simulink library "lib_SecCtrl_MASmsg"  (R2026a)
settings: Solver=VariableStepAuto
undefined symbols (not defined in the file): buses_lf, DiscIntNeverNeededParam, entity, iPs_lf, iQs_lf, last_send, m, Ps_lf, Qs_lf, set_DG_up, set_extra_satur, set_sending_cost, v_buses_mod
libraries: simulink x400, sl_discontinuities x10, eeGeneralControl x5
(part 9 of 12)

== system lib_SecCtrl_MASmsg/MAS messages/ID1/Send to neighbor1/five ==
  Message : Inport
  Cast1 : EntityMulticast  InputPortMessageModes=m  MulticastTag=ID2
  Cast1all : EntityMulticast  InputPortMessageModes=m  MulticastTag=ID2
  Cast2 : EntityMulticast  InputPortMessageModes=m  MulticastTag=ID2
  Cast2all : EntityMulticast  InputPortMessageModes=m  MulticastTag=ID2
  Cast3 : EntityMulticast  InputPortMessageModes=m  MulticastTag=ID0
  Cast3all : EntityMulticast  InputPortMessageModes=m  MulticastTag=ID0
  Cast4 : EntityMulticast  InputPortMessageModes=m  MulticastTag=ID0
  Cast4all : EntityMulticast  InputPortMessageModes=m  MulticastTag=ID0
  Cast5 : EntityMulticast  InputPortMessageModes=m  MulticastTag=ID0
  Cast5all : EntityMulticast  InputPortMessageModes=m  MulticastTag=ID0
  Entity Output Switch : EntityOutputSwitch  InputPortMessageModes=m  OutputPortMessageModes=m,m,m,m,m,m  NumberOutputPorts=6  SwitchingCriterion=From attribute  SwitchAttributeName=Select  InitialPortSelection=3
      settings: OutputPortMap=o0,o1,o2,o3,o4,o5
  Entity Replicator1 : EntityReplicator  InputPortMessageModes=m  OutputPortMessageModes=m,m,m,m,m  NumberReplicas=4
      settings: OutputPortMap=o0,o1,o2,o3,o4
  Entity Server : EntityServer  InputPortMessageModes=m  OutputPortMessageModes=m  Capacity=1  ServiceTimeValue=0  EntryAction=entity.Select = select(entity.Dest);
  select : Subsystem  TreatAsAtomicUnit=on
  wires:
  Entity Server/1 -> Entity Output Switch/1
  Entity Output Switch/5 -> Cast5/1
  Entity Output Switch/1 -> Cast1/1
  Entity Replicator1/3 -> Cast3all/1
  Entity Replicator1/4 -> Cast4all/1
  Entity Output Switch/3 -> Cast3/1
  Entity Output Switch/2 -> Cast2/1
  Entity Replicator1/2 -> Cast2all/1
  Entity Replicator1/1 -> Cast1all/1
  Message/1 -> Entity Server/1  "Message"
  Entity Replicator1/5 -> Cast5all/1
  Entity Output Switch/6 -> Entity Replicator1/1
  Entity Output Switch/4 -> Cast4/1

== system lib_SecCtrl_MASmsg/MAS messages/ID1/Send to neighbor1/four ==
  Message : Inport
  Cast1 : EntityMulticast  InputPortMessageModes=m  MulticastTag=ID1
  Cast1all : EntityMulticast  InputPortMessageModes=m  MulticastTag=ID1
  Cast2 : EntityMulticast  InputPortMessageModes=m  MulticastTag=ID3
  Cast2all : EntityMulticast  InputPortMessageModes=m  MulticastTag=ID3
  Cast3 : EntityMulticast  InputPortMessageModes=m  MulticastTag=ID0
  Cast3all : EntityMulticast  InputPortMessageModes=m  MulticastTag=ID0
  Cast4 : EntityMulticast  InputPortMessageModes=m  MulticastTag=ID0
  Cast4all : EntityMulticast  InputPortMessageModes=m  MulticastTag=ID0
  Entity Output Switch : EntityOutputSwitch  InputPortMessageModes=m  OutputPortMessageModes=m,m,m,m,m  NumberOutputPorts=5  SwitchingCriterion=From attribute  SwitchAttributeName=Select  InitialPortSelection=3
      settings: OutputPortMap=o0,o1,o2,o3,o4
  Entity Replicator1 : EntityReplicator  InputPortMessageModes=m  OutputPortMessageModes=m,m,m,m  NumberReplicas=3
      settings: OutputPortMap=o0,o1,o2,o3
  Entity Server : EntityServer  InputPortMessageModes=m  OutputPortMessageModes=m  Capacity=1  ServiceTimeValue=0  EntryAction=entity.Select = select(entity.Dest);
  select : Subsystem  TreatAsAtomicUnit=on
  wires:
  Entity Server/1 -> Entity Output Switch/1
  Message/1 -> Entity Server/1  "Message"
  Entity Output Switch/4 -> Cast4/1
  Entity Output Switch/2 -> Cast2/1
  Entity Replicator1/2 -> Cast2all/1
  Entity Replicator1/1 -> Cast1all/1
  Entity Output Switch/1 -> Cast1/1
  Entity Output Switch/3 -> Cast3/1
  Entity Output Switch/5 -> Entity Replicator1/1
  Entity Replicator1/4 -> Cast4all/1
  Entity Replicator1/3 -> Cast3all/1

== system lib_SecCtrl_MASmsg/MAS messages/ID1/Send to neighbor1/one ==
  Message : Inport
  Cast : EntityMulticast  InputPortMessageModes=m  MulticastTag=ID2
  Castall : EntityMulticast  InputPortMessageModes=m  MulticastTag=ID2
  Entity Output Switch1 : EntityOutputSwitch  InputPortMessageModes=m  OutputPortMessageModes=m,m  SwitchingCriterion=From attribute  SwitchAttributeName=Select  InitialPortSelection=3
  Entity Server : EntityServer  InputPortMessageModes=m  OutputPortMessageModes=m  Capacity=1  ServiceTimeValue=0  EntryAction=entity.Select = select(entity.Dest);
  select : Subsystem  TreatAsAtomicUnit=on
  wires:
  Message/1 -> Entity Server/1  "Message"
  Entity Server/1 -> Entity Output Switch1/1
  Entity Output Switch1/1 -> Cast/1
  Entity Output Switch1/2 -> Castall/1

== system lib_SecCtrl_MASmsg/MAS messages/ID1/Send to neighbor1/three ==
  Message : Inport
  Cast1 : EntityMulticast  InputPortMessageModes=m  MulticastTag=ID0
  Cast1all : EntityMulticast  InputPortMessageModes=m  MulticastTag=ID0
  Cast2 : EntityMulticast  InputPortMessageModes=m  MulticastTag=ID0
  Cast2all : EntityMulticast  InputPortMessageModes=m  MulticastTag=ID0
  Cast3 : EntityMulticast  InputPortMessageModes=m  MulticastTag=ID0
  Cast3all : EntityMulticast  InputPortMessageModes=m  MulticastTag=ID0
  Entity Output Switch : EntityOutputSwitch  InputPortMessageModes=m  OutputPortMessageModes=m,m,m,m  NumberOutputPorts=4  SwitchingCriterion=From attribute  SwitchAttributeName=Select  InitialPortSelection=3
      settings: OutputPortMap=o0,o1,o2,o3
  Entity Replicator1 : EntityReplicator  InputPortMessageModes=m  OutputPortMessageModes=m,m,m  NumberReplicas=2
      settings: OutputPortMap=o0,o1,o2
  Entity Server : EntityServer  InputPortMessageModes=m  OutputPortMessageModes=m  Capacity=1  ServiceTimeValue=0  EntryAction=entity.Select = select(entity.Dest);
  select : Subsystem  TreatAsAtomicUnit=on
  wires:
  Entity Server/1 -> Entity Output Switch/1
  Message/1 -> Entity Server/1  "Message"
  Entity Output Switch/3 -> Cast3/1
  Entity Replicator1/3 -> Cast3all/1
  Entity Output Switch/1 -> Cast1/1
  Entity Replicator1/1 -> Cast1all/1
  Entity Replicator1/2 -> Cast2all/1
  Entity Output Switch/2 -> Cast2/1
  Entity Output Switch/4 -> Entity Replicator1/1

== system lib_SecCtrl_MASmsg/MAS messages/ID1/Send to neighbor1/two ==
  Message : Inport
  Cast1 : EntityMulticast  InputPortMessageModes=m  MulticastTag=ID5
  Cast1all : EntityMulticast  InputPortMessageModes=m  MulticastTag=ID5
  Cast2 : EntityMulticast  InputPortMessageModes=m  MulticastTag=ID2
  Cast2all : EntityMulticast  InputPortMessageModes=m  MulticastTag=ID2
  Entity Output Switch : EntityOutputSwitch  InputPortMessageModes=m  OutputPortMessageModes=m,m,m  NumberOutputPorts=3  SwitchingCriterion=From attribute  SwitchAttributeName=Select  InitialPortSelection=3
      settings: OutputPortMap=o0,o1,o2
  Entity Replicator1 : EntityReplicator  InputPortMessageModes=m  OutputPortMessageModes=m,m
  Entity Server : EntityServer  InputPortMessageModes=m  OutputPortMessageModes=m  Capacity=1  ServiceTimeValue=0  EntryAction=entity.Select = select(entity.Dest);
  select : Subsystem  TreatAsAtomicUnit=on
  wires:
  Entity Server/1 -> Entity Output Switch/1
  Entity Output Switch/2 -> Cast2/1
  Entity Output Switch/1 -> Cast1/1
  Message/1 -> Entity Server/1  "Message"
  Entity Replicator1/1 -> Cast1all/1
  Entity Replicator1/2 -> Cast2all/1
  Entity Output Switch/3 -> Entity Replicator1/1

== system lib_SecCtrl_MASmsg/MAS messages/ID1/Send to neighbor2/five ==
  Message : Inport
  Cast1 : EntityMulticast  InputPortMessageModes=m  MulticastTag=ID2
  Cast1all : EntityMulticast  InputPortMessageModes=m  MulticastTag=ID2
  Cast2 : EntityMulticast  InputPortMessageModes=m  MulticastTag=ID2
  Cast2all : EntityMulticast  InputPortMessageModes=m  MulticastTag=ID2
  Cast3 : EntityMulticast  InputPortMessageModes=m  MulticastTag=ID0
  Cast3all : EntityMulticast  InputPortMessageModes=m  MulticastTag=ID0
  Cast4 : EntityMulticast  InputPortMessageModes=m  MulticastTag=ID0
  Cast4all : EntityMulticast  InputPortMessageModes=m  MulticastTag=ID0
  Cast5 : EntityMulticast  InputPortMessageModes=m  MulticastTag=ID0
  Cast5all : EntityMulticast  InputPortMessageModes=m  MulticastTag=ID0
  Entity Output Switch : EntityOutputSwitch  InputPortMessageModes=m  OutputPortMessageModes=m,m,m,m,m,m  NumberOutputPorts=6  SwitchingCriterion=From attribute  SwitchAttributeName=Select  InitialPortSelection=3
      settings: OutputPortMap=o0,o1,o2,o3,o4,o5
  Entity Replicator1 : EntityReplicator  InputPortMessageModes=m  OutputPortMessageModes=m,m,m,m,m  NumberReplicas=4
      settings: OutputPortMap=o0,o1,o2,o3,o4
  Entity Server : EntityServer  InputPortMessageModes=m  OutputPortMessageModes=m  Capacity=1  ServiceTimeValue=0  EntryAction=entity.Select = select(entity.Dest);
  select : Subsystem  TreatAsAtomicUnit=on
  wires:
  Entity Output Switch/4 -> Cast4/1
  Entity Output Switch/6 -> Entity Replicator1/1
  Entity Replicator1/5 -> Cast5all/1
  Message/1 -> Entity Server/1  "Message"
  Entity Replicator1/1 -> Cast1all/1
  Entity Replicator1/2 -> Cast2all/1
  Entity Output Switch/2 -> Cast2/1
  Entity Output Switch/3 -> Cast3/1
  Entity Replicator1/4 -> Cast4all/1
  Entity Replicator1/3 -> Cast3all/1
  Entity Output Switch/1 -> Cast1/1
  Entity Output Switch/5 -> Cast5/1
  Entity Server/1 -> Entity Output Switch/1

== system lib_SecCtrl_MASmsg/MAS messages/ID1/Send to neighbor2/four ==
  Message : Inport
  Cast1 : EntityMulticast  InputPortMessageModes=m  MulticastTag=ID1
  Cast1all : EntityMulticast  InputPortMessageModes=m  MulticastTag=ID1
  Cast2 : EntityMulticast  InputPortMessageModes=m  MulticastTag=ID3
  Cast2all : EntityMulticast  InputPortMessageModes=m  MulticastTag=ID3
  Cast3 : EntityMulticast  InputPortMessageModes=m  MulticastTag=ID0
  Cast3all : EntityMulticast  InputPortMessageModes=m  MulticastTag=ID0
  Cast4 : EntityMulticast  InputPortMessageModes=m  MulticastTag=ID0
  Cast4all : EntityMulticast  InputPortMessageModes=m  MulticastTag=ID0
  Entity Output Switch : EntityOutputSwitch  InputPortMessageModes=m  OutputPortMessageModes=m,m,m,m,m  NumberOutputPorts=5  SwitchingCriterion=From attribute  SwitchAttributeName=Select  InitialPortSelection=3
      settings: OutputPortMap=o0,o1,o2,o3,o4
  Entity Replicator1 : EntityReplicator  InputPortMessageModes=m  OutputPortMessageModes=m,m,m,m  NumberReplicas=3
      settings: OutputPortMap=o0,o1,o2,o3
  Entity Server : EntityServer  InputPortMessageModes=m  OutputPortMessageModes=m  Capacity=1  ServiceTimeValue=0  EntryAction=entity.Select = select(entity.Dest);
  select : Subsystem  TreatAsAtomicUnit=on
  wires:
  Entity Replicator1/3 -> Cast3all/1
  Entity Replicator1/4 -> Cast4all/1
  Entity Output Switch/5 -> Entity Replicator1/1
  Entity Output Switch/3 -> Cast3/1
  Entity Output Switch/1 -> Cast1/1
  Entity Replicator1/1 -> Cast1all/1
  Entity Replicator1/2 -> Cast2all/1
  Entity Output Switch/2 -> Cast2/1
  Entity Output Switch/4 -> Cast4/1
  Message/1 -> Entity Server/1  "Message"
  Entity Server/1 -> Entity Output Switch/1

== system lib_SecCtrl_MASmsg/MAS messages/ID1/Send to neighbor2/one ==
  Message : Inport
  Cast : EntityMulticast  InputPortMessageModes=m  MulticastTag=ID2
  Castall : EntityMulticast  InputPortMessageModes=m  MulticastTag=ID2
  Entity Output Switch1 : EntityOutputSwitch  InputPortMessageModes=m  OutputPortMessageModes=m,m  SwitchingCriterion=From attribute  SwitchAttributeName=Select  InitialPortSelection=3
  Entity Server : EntityServer  InputPortMessageModes=m  OutputPortMessageModes=m  Capacity=1  ServiceTimeValue=0  EntryAction=entity.Select = select(entity.Dest);
  select : Subsystem  TreatAsAtomicUnit=on
  wires:
  Entity Output Switch1/2 -> Castall/1
  Entity Output Switch1/1 -> Cast/1
  Entity Server/1 -> Entity Output Switch1/1
  Message/1 -> Entity Server/1  "Message"

== system lib_SecCtrl_MASmsg/MAS messages/ID1/Send to neighbor2/three ==
  Message : Inport
  Cast1 : EntityMulticast  InputPortMessageModes=m  MulticastTag=ID0
  Cast1all : EntityMulticast  InputPortMessageModes=m  MulticastTag=ID0
  Cast2 : EntityMulticast  InputPortMessageModes=m  MulticastTag=ID0
  Cast2all : EntityMulticast  InputPortMessageModes=m  MulticastTag=ID0
  Cast3 : EntityMulticast  InputPortMessageModes=m  MulticastTag=ID0
  Cast3all : EntityMulticast  InputPortMessageModes=m  MulticastTag=ID0
  Entity Output Switch : EntityOutputSwitch  InputPortMessageModes=m  OutputPortMessageModes=m,m,m,m  NumberOutputPorts=4  SwitchingCriterion=From attribute  SwitchAttributeName=Select  InitialPortSelection=3
      settings: OutputPortMap=o0,o1,o2,o3
  Entity Replicator1 : EntityReplicator  InputPortMessageModes=m  OutputPortMessageModes=m,m,m  NumberReplicas=2
      settings: OutputPortMap=o0,o1,o2
  Entity Server : EntityServer  InputPortMessageModes=m  OutputPortMessageModes=m  Capacity=1  ServiceTimeValue=0  EntryAction=entity.Select = select(entity.Dest);
  select : Subsystem  TreatAsAtomicUnit=on
  wires:
  Entity Output Switch/4 -> Entity Replicator1/1
  Entity Output Switch/2 -> Cast2/1
  Entity Replicator1/2 -> Cast2all/1
  Entity Replicator1/1 -> Cast1all/1
  Entity Output Switch/1 -> Cast1/1
  Entity Replicator1/3 -> Cast3all/1
  Entity Output Switch/3 -> Cast3/1
  Message/1 -> Entity Server/1  "Message"
  Entity Server/1 -> Entity Output Switch/1

== system lib_SecCtrl_MASmsg/MAS messages/ID1/Send to neighbor2/two ==
  Message : Inport
  Cast1 : EntityMulticast  InputPortMessageModes=m  MulticastTag=ID5
  Cast1all : EntityMulticast  InputPortMessageModes=m  MulticastTag=ID5
  Cast2 : EntityMulticast  InputPortMessageModes=m  MulticastTag=ID2
  Cast2all : EntityMulticast  InputPortMessageModes=m  MulticastTag=ID2
  Entity Output Switch : EntityOutputSwitch  InputPortMessageModes=m  OutputPortMessageModes=m,m,m  NumberOutputPorts=3  SwitchingCriterion=From attribute  SwitchAttributeName=Select  InitialPortSelection=3
      settings: OutputPortMap=o0,o1,o2
  Entity Replicator1 : EntityReplicator  InputPortMessageModes=m  OutputPortMessageModes=m,m
  Entity Server : EntityServer  InputPortMessageModes=m  OutputPortMessageModes=m  Capacity=1  ServiceTimeValue=0  EntryAction=entity.Select = select(entity.Dest);
  select : Subsystem  TreatAsAtomicUnit=on
  wires:
  Entity Output Switch/3 -> Entity Replicator1/1
  Entity Replicator1/2 -> Cast2all/1
  Entity Replicator1/1 -> Cast1all/1
  Message/1 -> Entity Server/1  "Message"
  Entity Output Switch/1 -> Cast1/1
  Entity Output Switch/2 -> Cast2/1
  Entity Server/1 -> Entity Output Switch/1

== system lib_SecCtrl_MASmsg/MAS messages/ID2/Send to neighbor/five ==
  Message : Inport
  Cast1 : EntityMulticast  InputPortMessageModes=m  MulticastTag=ID2
  Cast1all : EntityMulticast  InputPortMessageModes=m  MulticastTag=ID2
  Cast2 : EntityMulticast  InputPortMessageModes=m  MulticastTag=ID2
  Cast2all : EntityMulticast  InputPortMessageModes=m  MulticastTag=ID2
  Cast3 : EntityMulticast  InputPortMessageModes=m  MulticastTag=ID0
  Cast3all : EntityMulticast  InputPortMessageModes=m  MulticastTag=ID0
  Cast4 : EntityMulticast  InputPortMessageModes=m  MulticastTag=ID0
  Cast4all : EntityMulticast  InputPortMessageModes=m  MulticastTag=ID0
  Cast5 : EntityMulticast  InputPortMessageModes=m  MulticastTag=ID0
  Cast5all : EntityMulticast  InputPortMessageModes=m  MulticastTag=ID0
  Entity Output Switch : EntityOutputSwitch  InputPortMessageModes=m  OutputPortMessageModes=m,m,m,m,m,m  NumberOutputPorts=6  SwitchingCriterion=From attribute  SwitchAttributeName=Select  InitialPortSelection=3
      settings: OutputPortMap=o0,o1,o2,o3,o4,o5
  Entity Replicator1 : EntityReplicator  InputPortMessageModes=m  OutputPortMessageModes=m,m,m,m,m  NumberReplicas=4
      settings: OutputPortMap=o0,o1,o2,o3,o4
  Entity Server : EntityServer  InputPortMessageModes=m  OutputPortMessageModes=m  Capacity=1  ServiceTimeValue=0  EntryAction=entity.Select = select(entity.Dest);
  select : Subsystem  TreatAsAtomicUnit=on
  wires:
  Entity Server/1 -> Entity Output Switch/1
  Entity Output Switch/5 -> Cast5/1
  Entity Output Switch/1 -> Cast1/1
  Entity Replicator1/3 -> Cast3all/1
  Entity Replicator1/4 -> Cast4all/1
  Entity Output Switch/3 -> Cast3/1
  Entity Output Switch/2 -> Cast2/1
  Entity Replicator1/2 -> Cast2all/1
  Entity Replicator1/1 -> Cast1all/1
  Message/1 -> Entity Server/1  "Message"
  Entity Replicator1/5 -> Cast5all/1
  Entity Output Switch/6 -> Entity Replicator1/1
  Entity Output Switch/4 -> Cast4/1

== system lib_SecCtrl_MASmsg/MAS messages/ID2/Send to neighbor/four ==
  Message : Inport
  Cast1 : EntityMulticast  InputPortMessageModes=m  MulticastTag=ID1
  Cast1all : EntityMulticast  InputPortMessageModes=m  MulticastTag=ID1
  Cast2 : EntityMulticast  InputPortMessageModes=m  MulticastTag=ID3
  Cast2all : EntityMulticast  InputPortMessageModes=m  MulticastTag=ID3
  Cast3 : EntityMulticast  InputPortMessageModes=m  MulticastTag=ID0
  Cast3all : EntityMulticast  InputPortMessageModes=m  MulticastTag=ID0
  Cast4 : EntityMulticast  InputPortMessageModes=m  MulticastTag=ID0
  Cast4all : EntityMulticast  InputPortMessageModes=m  MulticastTag=ID0
  Entity Output Switch : EntityOutputSwitch  InputPortMessageModes=m  OutputPortMessageModes=m,m,m,m,m  NumberOutputPorts=5  SwitchingCriterion=From attribute  SwitchAttributeName=Select  InitialPortSelection=3
      settings: OutputPortMap=o0,o1,o2,o3,o4
  Entity Replicator1 : EntityReplicator  InputPortMessageModes=m  OutputPortMessageModes=m,m,m,m  NumberReplicas=3
      settings: OutputPortMap=o0,o1,o2,o3
  Entity Server : EntityServer  InputPortMessageModes=m  OutputPortMessageModes=m  Capacity=1  ServiceTimeValue=0  EntryAction=entity.Select = select(entity.Dest);
  select : Subsystem  TreatAsAtomicUnit=on
  wires:
  Entity Server/1 -> Entity Output Switch/1
  Message/1 -> Entity Server/1  "Message"
  Entity Output Switch/4 -> Cast4/1
  Entity Output Switch/2 -> Cast2/1
  Entity Replicator1/2 -> Cast2all/1
  Entity Replicator1/1 -> Cast1all/1
  Entity Output Switch/1 -> Cast1/1
  Entity Output Switch/3 -> Cast3/1
  Entity Output Switch/5 -> Entity Replicator1/1
  Entity Replicator1/4 -> Cast4all/1
  Entity Replicator1/3 -> Cast3all/1

== system lib_SecCtrl_MASmsg/MAS messages/ID2/Send to neighbor/one ==
  Message : Inport
  Cast : EntityMulticast  InputPortMessageModes=m  MulticastTag=ID2
  Castall : EntityMulticast  InputPortMessageModes=m  MulticastTag=ID2
  Entity Output Switch1 : EntityOutputSwitch  InputPortMessageModes=m  OutputPortMessageModes=m,m  SwitchingCriterion=From attribute  SwitchAttributeName=Select  InitialPortSelection=3
  Entity Server : EntityServer  InputPortMessageModes=m  OutputPortMessageModes=m  Capacity=1  ServiceTimeValue=0  EntryAction=entity.Select = select(entity.Dest);
  select : Subsystem  TreatAsAtomicUnit=on
  wires:
  Message/1 -> Entity Server/1  "Message"
  Entity Server/1 -> Entity Output Switch1/1
  Entity Output Switch1/1 -> Cast/1
  Entity Output Switch1/2 -> Castall/1

== system lib_SecCtrl_MASmsg/MAS messages/ID2/Send to neighbor/three ==
  Message : Inport
  Cast1 : EntityMulticast  InputPortMessageModes=m  MulticastTag=ID0
  Cast1all : EntityMulticast  InputPortMessageModes=m  MulticastTag=ID0
  Cast2 : EntityMulticast  InputPortMessageModes=m  MulticastTag=ID0
  Cast2all : EntityMulticast  InputPortMessageModes=m  MulticastTag=ID0
  Cast3 : EntityMulticast  InputPortMessageModes=m  MulticastTag=ID0
  Cast3all : EntityMulticast  InputPortMessageModes=m  MulticastTag=ID0
  Entity Output Switch : EntityOutputSwitch  InputPortMessageModes=m  OutputPortMessageModes=m,m,m,m  NumberOutputPorts=4  SwitchingCriterion=From attribute  SwitchAttributeName=Select  InitialPortSelection=3
      settings: OutputPortMap=o0,o1,o2,o3
  Entity Replicator1 : EntityReplicator  InputPortMessageModes=m  OutputPortMessageModes=m,m,m  NumberReplicas=2
      settings: OutputPortMap=o0,o1,o2
  Entity Server : EntityServer  InputPortMessageModes=m  OutputPortMessageModes=m  Capacity=1  ServiceTimeValue=0  EntryAction=entity.Select = select(entity.Dest);
  select : Subsystem  TreatAsAtomicUnit=on
  wires:
  Entity Server/1 -> Entity Output Switch/1
  Message/1 -> Entity Server/1  "Message"
  Entity Output Switch/3 -> Cast3/1
  Entity Replicator1/3 -> Cast3all/1
  Entity Output Switch/1 -> Cast1/1
  Entity Replicator1/1 -> Cast1all/1
  Entity Replicator1/2 -> Cast2all/1
  Entity Output Switch/2 -> Cast2/1
  Entity Output Switch/4 -> Entity Replicator1/1

== system lib_SecCtrl_MASmsg/MAS messages/ID2/Send to neighbor/two ==
  Message : Inport
  Cast1 : EntityMulticast  InputPortMessageModes=m  MulticastTag=ID1
  Cast1all : EntityMulticast  InputPortMessageModes=m  MulticastTag=ID1
  Cast2 : EntityMulticast  InputPortMessageModes=m  MulticastTag=ID3
  Cast2all : EntityMulticast  InputPortMessageModes=m  MulticastTag=ID3
  Entity Output Switch : EntityOutputSwitch  InputPortMessageModes=m  OutputPortMessageModes=m,m,m  NumberOutputPorts=3  SwitchingCriterion=From attribute  SwitchAttributeName=Select  InitialPortSelection=3
      settings: OutputPortMap=o0,o1,o2
  Entity Replicator1 : EntityReplicator  InputPortMessageModes=m  OutputPortMessageModes=m,m
  Entity Server : EntityServer  InputPortMessageModes=m  OutputPortMessageModes=m  Capacity=1  ServiceTimeValue=0  EntryAction=entity.Select = select(entity.Dest);
  select : Subsystem  TreatAsAtomicUnit=on
  wires:
  Entity Server/1 -> Entity Output Switch/1
  Entity Output Switch/2 -> Cast2/1
  Entity Output Switch/1 -> Cast1/1
  Message/1 -> Entity Server/1  "Message"
  Entity Replicator1/1 -> Cast1all/1
  Entity Replicator1/2 -> Cast2all/1
  Entity Output Switch/3 -> Entity Replicator1/1

== system lib_SecCtrl_MASmsg/MAS messages/ID2/Send to neighbor1/five ==
  Message : Inport
  Cast1 : EntityMulticast  InputPortMessageModes=m  MulticastTag=ID2
  Cast1all : EntityMulticast  InputPortMessageModes=m  MulticastTag=ID2
  Cast2 : EntityMulticast  InputPortMessageModes=m  MulticastTag=ID2
  Cast2all : EntityMulticast  InputPortMessageModes=m  MulticastTag=ID2
  Cast3 : EntityMulticast  InputPortMessageModes=m  MulticastTag=ID0
  Cast3all : EntityMulticast  InputPortMessageModes=m  MulticastTag=ID0
  Cast4 : EntityMulticast  InputPortMessageModes=m  MulticastTag=ID0
  Cast4all : EntityMulticast  InputPortMessageModes=m  MulticastTag=ID0
  Cast5 : EntityMulticast  InputPortMessageModes=m  MulticastTag=ID0
  Cast5all : EntityMulticast  InputPortMessageModes=m  MulticastTag=ID0
  Entity Output Switch : EntityOutputSwitch  InputPortMessageModes=m  OutputPortMessageModes=m,m,m,m,m,m  NumberOutputPorts=6  SwitchingCriterion=From attribute  SwitchAttributeName=Select  InitialPortSelection=3
      settings: OutputPortMap=o0,o1,o2,o3,o4,o5
  Entity Replicator1 : EntityReplicator  InputPortMessageModes=m  OutputPortMessageModes=m,m,m,m,m  NumberReplicas=4
      settings: OutputPortMap=o0,o1,o2,o3,o4
  Entity Server : EntityServer  InputPortMessageModes=m  OutputPortMessageModes=m  Capacity=1  ServiceTimeValue=0  EntryAction=entity.Select = select(entity.Dest);
  select : Subsystem  TreatAsAtomicUnit=on
  wires:
  Entity Output Switch/4 -> Cast4/1
  Entity Output Switch/6 -> Entity Replicator1/1
  Entity Replicator1/5 -> Cast5all/1
  Message/1 -> Entity Server/1  "Message"
  Entity Replicator1/1 -> Cast1all/1
  Entity Replicator1/2 -> Cast2all/1
  Entity Output Switch/2 -> Cast2/1
  Entity Output Switch/3 -> Cast3/1
  Entity Replicator1/4 -> Cast4all/1
  Entity Replicator1/3 -> Cast3all/1
  Entity Output Switch/1 -> Cast1/1
  Entity Output Switch/5 -> Cast5/1
  Entity Server/1 -> Entity Output Switch/1

== system lib_SecCtrl_MASmsg/MAS messages/ID2/Send to neighbor1/four ==
  Message : Inport
  Cast1 : EntityMulticast  InputPortMessageModes=m  MulticastTag=ID1
  Cast1all : EntityMulticast  InputPortMessageModes=m  MulticastTag=ID1
  Cast2 : EntityMulticast  InputPortMessageModes=m  MulticastTag=ID3
  Cast2all : EntityMulticast  InputPortMessageModes=m  MulticastTag=ID3
  Cast3 : EntityMulticast  InputPortMessageModes=m  MulticastTag=ID0
  Cast3all : EntityMulticast  InputPortMessageModes=m  MulticastTag=ID0
  Cast4 : EntityMulticast  InputPortMessageModes=m  MulticastTag=ID0
  Cast4all : EntityMulticast  InputPortMessageModes=m  MulticastTag=ID0
  Entity Output Switch : EntityOutputSwitch  InputPortMessageModes=m  OutputPortMessageModes=m,m,m,m,m  NumberOutputPorts=5  SwitchingCriterion=From attribute  SwitchAttributeName=Select  InitialPortSelection=3
      settings: OutputPortMap=o0,o1,o2,o3,o4
  Entity Replicator1 : EntityReplicator  InputPortMessageModes=m  OutputPortMessageModes=m,m,m,m  NumberReplicas=3
      settings: OutputPortMap=o0,o1,o2,o3
  Entity Server : EntityServer  InputPortMessageModes=m  OutputPortMessageModes=m  Capacity=1  ServiceTimeValue=0  EntryAction=entity.Select = select(entity.Dest);
  select : Subsystem  TreatAsAtomicUnit=on
  wires:
  Entity Replicator1/3 -> Cast3all/1
  Entity Replicator1/4 -> Cast4all/1
  Entity Output Switch/5 -> Entity Replicator1/1
  Entity Output Switch/3 -> Cast3/1
  Entity Output Switch/1 -> Cast1/1
  Entity Replicator1/1 -> Cast1all/1
  Entity Replicator1/2 -> Cast2all/1
  Entity Output Switch/2 -> Cast2/1
  Entity Output Switch/4 -> Cast4/1
  Message/1 -> Entity Server/1  "Message"
  Entity Server/1 -> Entity Output Switch/1

== system lib_SecCtrl_MASmsg/MAS messages/ID2/Send to neighbor1/one ==
  Message : Inport
  Cast : EntityMulticast  InputPortMessageModes=m  MulticastTag=ID2
  Castall : EntityMulticast  InputPortMessageModes=m  MulticastTag=ID2
  Entity Output Switch1 : EntityOutputSwitch  InputPortMessageModes=m  OutputPortMessageModes=m,m  SwitchingCriterion=From attribute  SwitchAttributeName=Select  InitialPortSelection=3
  Entity Server : EntityServer  InputPortMessageModes=m  OutputPortMessageModes=m  Capacity=1  ServiceTimeValue=0  EntryAction=entity.Select = select(entity.Dest);
  select : Subsystem  TreatAsAtomicUnit=on
  wires:
  Entity Output Switch1/2 -> Castall/1
  Entity Output Switch1/1 -> Cast/1
  Entity Server/1 -> Entity Output Switch1/1
  Message/1 -> Entity Server/1  "Message"

== system lib_SecCtrl_MASmsg/MAS messages/ID2/Send to neighbor1/three ==
  Message : Inport
  Cast1 : EntityMulticast  InputPortMessageModes=m  MulticastTag=ID0
  Cast1all : EntityMulticast  InputPortMessageModes=m  MulticastTag=ID0
  Cast2 : EntityMulticast  InputPortMessageModes=m  MulticastTag=ID0
  Cast2all : EntityMulticast  InputPortMessageModes=m  MulticastTag=ID0
  Cast3 : EntityMulticast  InputPortMessageModes=m  MulticastTag=ID0
  Cast3all : EntityMulticast  InputPortMessageModes=m  MulticastTag=ID0
  Entity Output Switch : EntityOutputSwitch  InputPortMessageModes=m  OutputPortMessageModes=m,m,m,m  NumberOutputPorts=4  SwitchingCriterion=From attribute  SwitchAttributeName=Select  InitialPortSelection=3
      settings: OutputPortMap=o0,o1,o2,o3
  Entity Replicator1 : EntityReplicator  InputPortMessageModes=m  OutputPortMessageModes=m,m,m  NumberReplicas=2
      settings: OutputPortMap=o0,o1,o2
  Entity Server : EntityServer  InputPortMessageModes=m  OutputPortMessageModes=m  Capacity=1  ServiceTimeValue=0  EntryAction=entity.Select = select(entity.Dest);
  select : Subsystem  TreatAsAtomicUnit=on
  wires:
  Entity Output Switch/4 -> Entity Replicator1/1
  Entity Output Switch/2 -> Cast2/1
  Entity Replicator1/2 -> Cast2all/1
  Entity Replicator1/1 -> Cast1all/1
  Entity Output Switch/1 -> Cast1/1
  Entity Replicator1/3 -> Cast3all/1
  Entity Output Switch/3 -> Cast3/1
  Message/1 -> Entity Server/1  "Message"
  Entity Server/1 -> Entity Output Switch/1

== system lib_SecCtrl_MASmsg/MAS messages/ID2/Send to neighbor1/two ==
  Message : Inport
  Cast1 : EntityMulticast  InputPortMessageModes=m  MulticastTag=ID1
  Cast1all : EntityMulticast  InputPortMessageModes=m  MulticastTag=ID1
  Cast2 : EntityMulticast  InputPortMessageModes=m  MulticastTag=ID3
  Cast2all : EntityMulticast  InputPortMessageModes=m  MulticastTag=ID3
  Entity Output Switch : EntityOutputSwitch  InputPortMessageModes=m  OutputPortMessageModes=m,m,m  NumberOutputPorts=3  SwitchingCriterion=From attribute  SwitchAttributeName=Select  InitialPortSelection=3
      settings: OutputPortMap=o0,o1,o2
  Entity Replicator1 : EntityReplicator  InputPortMessageModes=m  OutputPortMessageModes=m,m
  Entity Server : EntityServer  InputPortMessageModes=m  OutputPortMessageModes=m  Capacity=1  ServiceTimeValue=0  EntryAction=entity.Select = select(entity.Dest);
  select : Subsystem  TreatAsAtomicUnit=on
  wires:
  Entity Output Switch/3 -> Entity Replicator1/1
  Entity Replicator1/2 -> Cast2all/1
  Entity Replicator1/1 -> Cast1all/1
  Message/1 -> Entity Server/1  "Message"
  Entity Output Switch/1 -> Cast1/1
  Entity Output Switch/2 -> Cast2/1
  Entity Server/1 -> Entity Output Switch/1

== system lib_SecCtrl_MASmsg/MAS messages/ID2/Send to neighbor2/five ==
  Message : Inport
  Cast1 : EntityMulticast  InputPortMessageModes=m  MulticastTag=ID2
  Cast1all : EntityMulticast  InputPortMessageModes=m  MulticastTag=ID2
  Cast2 : EntityMulticast  InputPortMessageModes=m  MulticastTag=ID2
  Cast2all : EntityMulticast  InputPortMessageModes=m  MulticastTag=ID2
  Cast3 : EntityMulticast  InputPortMessageModes=m  MulticastTag=ID0
  Cast3all : EntityMulticast  InputPortMessageModes=m  MulticastTag=ID0
  Cast4 : EntityMulticast  InputPortMessageModes=m  MulticastTag=ID0
  Cast4all : EntityMulticast  InputPortMessageModes=m  MulticastTag=ID0
  Cast5 : EntityMulticast  InputPortMessageModes=m  MulticastTag=ID0
  Cast5all : EntityMulticast  InputPortMessageModes=m  MulticastTag=ID0
  Entity Output Switch : EntityOutputSwitch  InputPortMessageModes=m  OutputPortMessageModes=m,m,m,m,m,m  NumberOutputPorts=6  SwitchingCriterion=From attribute  SwitchAttributeName=Select  InitialPortSelection=3
      settings: OutputPortMap=o0,o1,o2,o3,o4,o5
  Entity Replicator1 : EntityReplicator  InputPortMessageModes=m  OutputPortMessageModes=m,m,m,m,m  NumberReplicas=4
      settings: OutputPortMap=o0,o1,o2,o3,o4
  Entity Server : EntityServer  InputPortMessageModes=m  OutputPortMessageModes=m  Capacity=1  ServiceTimeValue=0  EntryAction=entity.Select = select(entity.Dest);
  select : Subsystem  TreatAsAtomicUnit=on
  wires:
  Entity Server/1 -> Entity Output Switch/1
  Entity Output Switch/5 -> Cast5/1
  Entity Output Switch/1 -> Cast1/1
  Entity Replicator1/3 -> Cast3all/1
  Entity Replicator1/4 -> Cast4all/1
  Entity Output Switch/3 -> Cast3/1
  Entity Output Switch/2 -> Cast2/1
  Entity Replicator1/2 -> Cast2all/1
  Entity Replicator1/1 -> Cast1all/1
  Message/1 -> Entity Server/1  "Message"
  Entity Replicator1/5 -> Cast5all/1
  Entity Output Switch/6 -> Entity Replicator1/1
  Entity Output Switch/4 -> Cast4/1

== system lib_SecCtrl_MASmsg/MAS messages/ID2/Send to neighbor2/four ==
  Message : Inport
  Cast1 : EntityMulticast  InputPortMessageModes=m  MulticastTag=ID1
  Cast1all : EntityMulticast  InputPortMessageModes=m  MulticastTag=ID1
  Cast2 : EntityMulticast  InputPortMessageModes=m  MulticastTag=ID3
  Cast2all : EntityMulticast  InputPortMessageModes=m  MulticastTag=ID3
  Cast3 : EntityMulticast  InputPortMessageModes=m  MulticastTag=ID0
  Cast3all : EntityMulticast  InputPortMessageModes=m  MulticastTag=ID0
  Cast4 : EntityMulticast  InputPortMessageModes=m  MulticastTag=ID0
  Cast4all : EntityMulticast  InputPortMessageModes=m  MulticastTag=ID0
  Entity Output Switch : EntityOutputSwitch  InputPortMessageModes=m  OutputPortMessageModes=m,m,m,m,m  NumberOutputPorts=5  SwitchingCriterion=From attribute  SwitchAttributeName=Select  InitialPortSelection=3
      settings: OutputPortMap=o0,o1,o2,o3,o4
  Entity Replicator1 : EntityReplicator  InputPortMessageModes=m  OutputPortMessageModes=m,m,m,m  NumberReplicas=3
      settings: OutputPortMap=o0,o1,o2,o3
  Entity Server : EntityServer  InputPortMessageModes=m  OutputPortMessageModes=m  Capacity=1  ServiceTimeValue=0  EntryAction=entity.Select = select(entity.Dest);
  select : Subsystem  TreatAsAtomicUnit=on
  wires:
  Entity Server/1 -> Entity Output Switch/1
  Message/1 -> Entity Server/1  "Message"
  Entity Output Switch/4 -> Cast4/1
  Entity Output Switch/2 -> Cast2/1
  Entity Replicator1/2 -> Cast2all/1
  Entity Replicator1/1 -> Cast1all/1
  Entity Output Switch/1 -> Cast1/1
  Entity Output Switch/3 -> Cast3/1
  Entity Output Switch/5 -> Entity Replicator1/1
  Entity Replicator1/4 -> Cast4all/1
  Entity Replicator1/3 -> Cast3all/1

== system lib_SecCtrl_MASmsg/MAS messages/ID2/Send to neighbor2/one ==
  Message : Inport
  Cast : EntityMulticast  InputPortMessageModes=m  MulticastTag=ID2
  Castall : EntityMulticast  InputPortMessageModes=m  MulticastTag=ID2
  Entity Output Switch1 : EntityOutputSwitch  InputPortMessageModes=m  OutputPortMessageModes=m,m  SwitchingCriterion=From attribute  SwitchAttributeName=Select  InitialPortSelection=3
  Entity Server : EntityServer  InputPortMessageModes=m  OutputPortMessageModes=m  Capacity=1  ServiceTimeValue=0  EntryAction=entity.Select = select(entity.Dest);
  select : Subsystem  TreatAsAtomicUnit=on
  wires:
  Message/1 -> Entity Server/1  "Message"
  Entity Server/1 -> Entity Output Switch1/1
  Entity Output Switch1/1 -> Cast/1
  Entity Output Switch1/2 -> Castall/1

== system lib_SecCtrl_MASmsg/MAS messages/ID2/Send to neighbor2/three ==
  Message : Inport
  Cast1 : EntityMulticast  InputPortMessageModes=m  MulticastTag=ID0
  Cast1all : EntityMulticast  InputPortMessageModes=m  MulticastTag=ID0
  Cast2 : EntityMulticast  InputPortMessageModes=m  MulticastTag=ID0
  Cast2all : EntityMulticast  InputPortMessageModes=m  MulticastTag=ID0
  Cast3 : EntityMulticast  InputPortMessageModes=m  MulticastTag=ID0
  Cast3all : EntityMulticast  InputPortMessageModes=m  MulticastTag=ID0
  Entity Output Switch : EntityOutputSwitch  InputPortMessageModes=m  OutputPortMessageModes=m,m,m,m  NumberOutputPorts=4  SwitchingCriterion=From attribute  SwitchAttributeName=Select  InitialPortSelection=3
      settings: OutputPortMap=o0,o1,o2,o3
  Entity Replicator1 : EntityReplicator  InputPortMessageModes=m  OutputPortMessageModes=m,m,m  NumberReplicas=2
      settings: OutputPortMap=o0,o1,o2
  Entity Server : EntityServer  InputPortMessageModes=m  OutputPortMessageModes=m  Capacity=1  ServiceTimeValue=0  EntryAction=entity.Select = select(entity.Dest);
  select : Subsystem  TreatAsAtomicUnit=on
  wires:
  Entity Server/1 -> Entity Output Switch/1
  Message/1 -> Entity Server/1  "Message"
  Entity Output Switch/3 -> Cast3/1
  Entity Replicator1/3 -> Cast3all/1
  Entity Output Switch/1 -> Cast1/1
  Entity Replicator1/1 -> Cast1all/1
  Entity Replicator1/2 -> Cast2all/1
  Entity Output Switch/2 -> Cast2/1
  Entity Output Switch/4 -> Entity Replicator1/1

== system lib_SecCtrl_MASmsg/MAS messages/ID2/Send to neighbor2/two ==
  Message : Inport
  Cast1 : EntityMulticast  InputPortMessageModes=m  MulticastTag=ID1
  Cast1all : EntityMulticast  InputPortMessageModes=m  MulticastTag=ID1
  Cast2 : EntityMulticast  InputPortMessageModes=m  MulticastTag=ID3
  Cast2all : EntityMulticast  InputPortMessageModes=m  MulticastTag=ID3
  Entity Output Switch : EntityOutputSwitch  InputPortMessageModes=m  OutputPortMessageModes=m,m,m  NumberOutputPorts=3  SwitchingCriterion=From attribute  SwitchAttributeName=Select  InitialPortSelection=3
      settings: OutputPortMap=o0,o1,o2
  Entity Replicator1 : EntityReplicator  InputPortMessageModes=m  OutputPortMessageModes=m,m
  Entity Server : EntityServer  InputPortMessageModes=m  OutputPortMessageModes=m  Capacity=1  ServiceTimeValue=0  EntryAction=entity.Select = select(entity.Dest);
  select : Subsystem  TreatAsAtomicUnit=on
  wires:
  Entity Server/1 -> Entity Output Switch/1
  Entity Output Switch/2 -> Cast2/1
  Entity Output Switch/1 -> Cast1/1
  Message/1 -> Entity Server/1  "Message"
  Entity Replicator1/1 -> Cast1all/1
  Entity Replicator1/2 -> Cast2all/1
  Entity Output Switch/3 -> Entity Replicator1/1

== system lib_SecCtrl_MASmsg/MAS messages/ID3/Send to neighbor/five ==
  Message : Inport
  Cast1 : EntityMulticast  InputPortMessageModes=m  MulticastTag=ID2
  Cast1all : EntityMulticast  InputPortMessageModes=m  MulticastTag=ID2
  Cast2 : EntityMulticast  InputPortMessageModes=m  MulticastTag=ID2
  Cast2all : EntityMulticast  InputPortMessageModes=m  MulticastTag=ID2
  Cast3 : EntityMulticast  InputPortMessageModes=m  MulticastTag=ID0
  Cast3all : EntityMulticast  InputPortMessageModes=m  MulticastTag=ID0
  Cast4 : EntityMulticast  InputPortMessageModes=m  MulticastTag=ID0
  Cast4all : EntityMulticast  InputPortMessageModes=m  MulticastTag=ID0
  Cast5 : EntityMulticast  InputPortMessageModes=m  MulticastTag=ID0
  Cast5all : EntityMulticast  InputPortMessageModes=m  MulticastTag=ID0
  Entity Output Switch : EntityOutputSwitch  InputPortMessageModes=m  OutputPortMessageModes=m,m,m,m,m,m  NumberOutputPorts=6  SwitchingCriterion=From attribute  SwitchAttributeName=Select  InitialPortSelection=3
      settings: OutputPortMap=o0,o1,o2,o3,o4,o5
  Entity Replicator1 : EntityReplicator  InputPortMessageModes=m  OutputPortMessageModes=m,m,m,m,m  NumberReplicas=4
      settings: OutputPortMap=o0,o1,o2,o3,o4
  Entity Server : EntityServer  InputPortMessageModes=m  OutputPortMessageModes=m  Capacity=1  ServiceTimeValue=0  EntryAction=entity.Select = select(entity.Dest);
  select : Subsystem  TreatAsAtomicUnit=on
  wires:
  Entity Server/1 -> Entity Output Switch/1
  Entity Output Switch/5 -> Cast5/1
  Entity Output Switch/1 -> Cast1/1
  Entity Replicator1/3 -> Cast3all/1
  Entity Replicator1/4 -> Cast4all/1
  Entity Output Switch/3 -> Cast3/1
  Entity Output Switch/2 -> Cast2/1
  Entity Replicator1/2 -> Cast2all/1
  Entity Replicator1/1 -> Cast1all/1
  Message/1 -> Entity Server/1  "Message"
  Entity Replicator1/5 -> Cast5all/1
  Entity Output Switch/6 -> Entity Replicator1/1
  Entity Output Switch/4 -> Cast4/1

== system lib_SecCtrl_MASmsg/MAS messages/ID3/Send to neighbor/four ==
  Message : Inport
  Cast1 : EntityMulticast  InputPortMessageModes=m  MulticastTag=ID1
  Cast1all : EntityMulticast  InputPortMessageModes=m  MulticastTag=ID1
  Cast2 : EntityMulticast  InputPortMessageModes=m  MulticastTag=ID3
  Cast2all : EntityMulticast  InputPortMessageModes=m  MulticastTag=ID3
  Cast3 : EntityMulticast  InputPortMessageModes=m  MulticastTag=ID0
  Cast3all : EntityMulticast  InputPortMessageModes=m  MulticastTag=ID0
  Cast4 : EntityMulticast  InputPortMessageModes=m  MulticastTag=ID0
  Cast4all : EntityMulticast  InputPortMessageModes=m  MulticastTag=ID0
  Entity Output Switch : EntityOutputSwitch  InputPortMessageModes=m  OutputPortMessageModes=m,m,m,m,m  NumberOutputPorts=5  SwitchingCriterion=From attribute  SwitchAttributeName=Select  InitialPortSelection=3
      settings: OutputPortMap=o0,o1,o2,o3,o4
  Entity Replicator1 : EntityReplicator  InputPortMessageModes=m  OutputPortMessageModes=m,m,m,m  NumberReplicas=3
      settings: OutputPortMap=o0,o1,o2,o3
  Entity Server : EntityServer  InputPortMessageModes=m  OutputPortMessageModes=m  Capacity=1  ServiceTimeValue=0  EntryAction=entity.Select = select(entity.Dest);
  select : Subsystem  TreatAsAtomicUnit=on
  wires:
  Entity Server/1 -> Entity Output Switch/1
  Message/1 -> Entity Server/1  "Message"
  Entity Output Switch/4 -> Cast4/1
  Entity Output Switch/2 -> Cast2/1
  Entity Replicator1/2 -> Cast2all/1
  Entity Replicator1/1 -> Cast1all/1
  Entity Output Switch/1 -> Cast1/1
  Entity Output Switch/3 -> Cast3/1
  Entity Output Switch/5 -> Entity Replicator1/1
  Entity Replicator1/4 -> Cast4all/1
  Entity Replicator1/3 -> Cast3all/1

== system lib_SecCtrl_MASmsg/MAS messages/ID3/Send to neighbor/one ==
  Message : Inport
  Cast : EntityMulticast  InputPortMessageModes=m  MulticastTag=ID2
  Castall : EntityMulticast  InputPortMessageModes=m  MulticastTag=ID2
  Entity Output Switch1 : EntityOutputSwitch  InputPortMessageModes=m  OutputPortMessageModes=m,m  SwitchingCriterion=From attribute  SwitchAttributeName=Select  InitialPortSelection=3
  Entity Server : EntityServer  InputPortMessageModes=m  OutputPortMessageModes=m  Capacity=1  ServiceTimeValue=0  EntryAction=entity.Select = select(entity.Dest);
  select : Subsystem  TreatAsAtomicUnit=on
  wires:
  Message/1 -> Entity Server/1  "Message"
  Entity Server/1 -> Entity Output Switch1/1
  Entity Output Switch1/1 -> Cast/1
  Entity Output Switch1/2 -> Castall/1

== system lib_SecCtrl_MASmsg/MAS messages/ID3/Send to neighbor/three ==
  Message : Inport
  Cast1 : EntityMulticast  InputPortMessageModes=m  MulticastTag=ID0
  Cast1all : EntityMulticast  InputPortMessageModes=m  MulticastTag=ID0
  Cast2 : EntityMulticast  InputPortMessageModes=m  MulticastTag=ID0
  Cast2all : EntityMulticast  InputPortMessageModes=m  MulticastTag=ID0
  Cast3 : EntityMulticast  InputPortMessageModes=m  MulticastTag=ID0
  Cast3all : EntityMulticast  InputPortMessageModes=m  MulticastTag=ID0
  Entity Output Switch : EntityOutputSwitch  InputPortMessageModes=m  OutputPortMessageModes=m,m,m,m  NumberOutputPorts=4  SwitchingCriterion=From attribute  SwitchAttributeName=Select  InitialPortSelection=3
      settings: OutputPortMap=o0,o1,o2,o3
  Entity Replicator1 : EntityReplicator  InputPortMessageModes=m  OutputPortMessageModes=m,m,m  NumberReplicas=2
      settings: OutputPortMap=o0,o1,o2
  Entity Server : EntityServer  InputPortMessageModes=m  OutputPortMessageModes=m  Capacity=1  ServiceTimeValue=0  EntryAction=entity.Select = select(entity.Dest);
  select : Subsystem  TreatAsAtomicUnit=on
  wires:
  Entity Server/1 -> Entity Output Switch/1
  Message/1 -> Entity Server/1  "Message"
  Entity Output Switch/3 -> Cast3/1
  Entity Replicator1/3 -> Cast3all/1
  Entity Output Switch/1 -> Cast1/1
  Entity Replicator1/1 -> Cast1all/1
  Entity Replicator1/2 -> Cast2all/1
  Entity Output Switch/2 -> Cast2/1
  Entity Output Switch/4 -> Entity Replicator1/1

== system lib_SecCtrl_MASmsg/MAS messages/ID3/Send to neighbor/two ==
  Message : Inport
  Cast1 : EntityMulticast  InputPortMessageModes=m  MulticastTag=ID2
  Cast1all : EntityMulticast  InputPortMessageModes=m  MulticastTag=ID2
  Cast2 : EntityMulticast  InputPortMessageModes=m  MulticastTag=ID4
  Cast2all : EntityMulticast  InputPortMessageModes=m  MulticastTag=ID4
  Entity Output Switch : EntityOutputSwitch  InputPortMessageModes=m  OutputPortMessageModes=m,m,m  NumberOutputPorts=3  SwitchingCriterion=From attribute  SwitchAttributeName=Select  InitialPortSelection=3
      settings: OutputPortMap=o0,o1,o2
  Entity Replicator1 : EntityReplicator  InputPortMessageModes=m  OutputPortMessageModes=m,m
  Entity Server : EntityServer  InputPortMessageModes=m  OutputPortMessageModes=m  Capacity=1  ServiceTimeValue=0  EntryAction=entity.Select = select(entity.Dest);
  select : Subsystem  TreatAsAtomicUnit=on
  wires:
  Entity Server/1 -> Entity Output Switch/1
  Entity Output Switch/2 -> Cast2/1
  Entity Output Switch/1 -> Cast1/1
  Message/1 -> Entity Server/1  "Message"
  Entity Replicator1/1 -> Cast1all/1
  Entity Replicator1/2 -> Cast2all/1
  Entity Output Switch/3 -> Entity Replicator1/1

== system lib_SecCtrl_MASmsg/MAS messages/ID3/Send to neighbor1/five ==
  Message : Inport
  Cast1 : EntityMulticast  InputPortMessageModes=m  MulticastTag=ID2
  Cast1all : EntityMulticast  InputPortMessageModes=m  MulticastTag=ID2
  Cast2 : EntityMulticast  InputPortMessageModes=m  MulticastTag=ID2
  Cast2all : EntityMulticast  InputPortMessageModes=m  MulticastTag=ID2
  Cast3 : EntityMulticast  InputPortMessageModes=m  MulticastTag=ID0
  Cast3all : EntityMulticast  InputPortMessageModes=m  MulticastTag=ID0
  Cast4 : EntityMulticast  InputPortMessageModes=m  MulticastTag=ID0
  Cast4all : EntityMulticast  InputPortMessageModes=m  MulticastTag=ID0
  Cast5 : EntityMulticast  InputPortMessageModes=m  MulticastTag=ID0
  Cast5all : EntityMulticast  InputPortMessageModes=m  MulticastTag=ID0
  Entity Output Switch : EntityOutputSwitch  InputPortMessageModes=m  OutputPortMessageModes=m,m,m,m,m,m  NumberOutputPorts=6  SwitchingCriterion=From attribute  SwitchAttributeName=Select  InitialPortSelection=3
      settings: OutputPortMap=o0,o1,o2,o3,o4,o5
  Entity Replicator1 : EntityReplicator  InputPortMessageModes=m  OutputPortMessageModes=m,m,m,m,m  NumberReplicas=4
      settings: OutputPortMap=o0,o1,o2,o3,o4
  Entity Server : EntityServer  InputPortMessageModes=m  OutputPortMessageModes=m  Capacity=1  ServiceTimeValue=0  EntryAction=entity.Select = select(entity.Dest);
  select : Subsystem  TreatAsAtomicUnit=on
  wires:
  Entity Output Switch/4 -> Cast4/1
  Entity Output Switch/6 -> Entity Replicator1/1
  Entity Replicator1/5 -> Cast5all/1
  Message/1 -> Entity Server/1  "Message"
  Entity Replicator1/1 -> Cast1all/1
  Entity Replicator1/2 -> Cast2all/1
  Entity Output Switch/2 -> Cast2/1
  Entity Output Switch/3 -> Cast3/1
  Entity Replicator1/4 -> Cast4all/1
  Entity Replicator1/3 -> Cast3all/1
  Entity Output Switch/1 -> Cast1/1
  Entity Output Switch/5 -> Cast5/1
  Entity Server/1 -> Entity Output Switch/1

== system lib_SecCtrl_MASmsg/MAS messages/ID3/Send to neighbor1/four ==
  Message : Inport
  Cast1 : EntityMulticast  InputPortMessageModes=m  MulticastTag=ID1
  Cast1all : EntityMulticast  InputPortMessageModes=m  MulticastTag=ID1
  Cast2 : EntityMulticast  InputPortMessageModes=m  MulticastTag=ID3
  Cast2all : EntityMulticast  InputPortMessageModes=m  MulticastTag=ID3
  Cast3 : EntityMulticast  InputPortMessageModes=m  MulticastTag=ID0
  Cast3all : EntityMulticast  InputPortMessageModes=m  MulticastTag=ID0
  Cast4 : EntityMulticast  InputPortMessageModes=m  MulticastTag=ID0
  Cast4all : EntityMulticast  InputPortMessageModes=m  MulticastTag=ID0
  Entity Output Switch : EntityOutputSwitch  InputPortMessageModes=m  OutputPortMessageModes=m,m,m,m,m  NumberOutputPorts=5  SwitchingCriterion=From attribute  SwitchAttributeName=Select  InitialPortSelection=3
      settings: OutputPortMap=o0,o1,o2,o3,o4
  Entity Replicator1 : EntityReplicator  InputPortMessageModes=m  OutputPortMessageModes=m,m,m,m  NumberReplicas=3
      settings: OutputPortMap=o0,o1,o2,o3
  Entity Server : EntityServer  InputPortMessageModes=m  OutputPortMessageModes=m  Capacity=1  ServiceTimeValue=0  EntryAction=entity.Select = select(entity.Dest);
  select : Subsystem  TreatAsAtomicUnit=on
  wires:
  Entity Replicator1/3 -> Cast3all/1
  Entity Replicator1/4 -> Cast4all/1
  Entity Output Switch/5 -> Entity Replicator1/1
  Entity Output Switch/3 -> Cast3/1
  Entity Output Switch/1 -> Cast1/1
  Entity Replicator1/1 -> Cast1all/1
  Entity Replicator1/2 -> Cast2all/1
  Entity Output Switch/2 -> Cast2/1
  Entity Output Switch/4 -> Cast4/1
  Message/1 -> Entity Server/1  "Message"
  Entity Server/1 -> Entity Output Switch/1

== system lib_SecCtrl_MASmsg/MAS messages/ID3/Send to neighbor1/one ==
  Message : Inport
  Cast : EntityMulticast  InputPortMessageModes=m  MulticastTag=ID2
  Castall : EntityMulticast  InputPortMessageModes=m  MulticastTag=ID2
  Entity Output Switch1 : EntityOutputSwitch  InputPortMessageModes=m  OutputPortMessageModes=m,m  SwitchingCriterion=From attribute  SwitchAttributeName=Select  InitialPortSelection=3
  Entity Server : EntityServer  InputPortMessageModes=m  OutputPortMessageModes=m  Capacity=1  ServiceTimeValue=0  EntryAction=entity.Select = select(entity.Dest);
  select : Subsystem  TreatAsAtomicUnit=on
  wires:
  Entity Output Switch1/2 -> Castall/1
  Entity Output Switch1/1 -> Cast/1
  Entity Server/1 -> Entity Output Switch1/1
  Message/1 -> Entity Server/1  "Message"

== system lib_SecCtrl_MASmsg/MAS messages/ID3/Send to neighbor1/three ==
  Message : Inport
  Cast1 : EntityMulticast  InputPortMessageModes=m  MulticastTag=ID0
  Cast1all : EntityMulticast  InputPortMessageModes=m  MulticastTag=ID0
  Cast2 : EntityMulticast  InputPortMessageModes=m  MulticastTag=ID0
  Cast2all : EntityMulticast  InputPortMessageModes=m  MulticastTag=ID0
  Cast3 : EntityMulticast  InputPortMessageModes=m  MulticastTag=ID0
  Cast3all : EntityMulticast  InputPortMessageModes=m  MulticastTag=ID0
  Entity Output Switch : EntityOutputSwitch  InputPortMessageModes=m  OutputPortMessageModes=m,m,m,m  NumberOutputPorts=4  SwitchingCriterion=From attribute  SwitchAttributeName=Select  InitialPortSelection=3
      settings: OutputPortMap=o0,o1,o2,o3
  Entity Replicator1 : EntityReplicator  InputPortMessageModes=m  OutputPortMessageModes=m,m,m  NumberReplicas=2
      settings: OutputPortMap=o0,o1,o2
  Entity Server : EntityServer  InputPortMessageModes=m  OutputPortMessageModes=m  Capacity=1  ServiceTimeValue=0  EntryAction=entity.Select = select(entity.Dest);
  select : Subsystem  TreatAsAtomicUnit=on
  wires:
  Entity Output Switch/4 -> Entity Replicator1/1
  Entity Output Switch/2 -> Cast2/1
  Entity Replicator1/2 -> Cast2all/1
  Entity Replicator1/1 -> Cast1all/1
  Entity Output Switch/1 -> Cast1/1
  Entity Replicator1/3 -> Cast3all/1
  Entity Output Switch/3 -> Cast3/1
  Message/1 -> Entity Server/1  "Message"
  Entity Server/1 -> Entity Output Switch/1
